simulink subsystem "FanModule_2025a"  (R2026a)
settings: Solver=VariableStepAuto
model mask{min_fan_speed=0.05, tau=0.1, max_thrust=3.53, radius=0.5, max_speed=62500}
  mask prompts: min_fan_speed "min Fan Speed (%)"; tau "Time Constant (s)"; max_thrust "Max Thrust (N)"; radius "Radius (m)"; max_speed "Max Speed (RPM)"
undefined symbols (not defined in the file): IN
settings Model: Creator=wangzerun  LastModifiedBy=asing

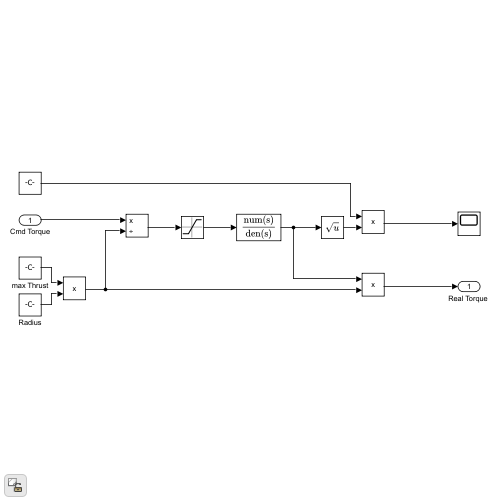
[thumbnail: Simulink's stored preview of the top-level diagram]
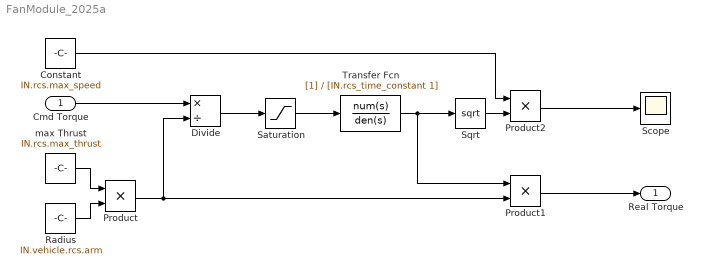
== system FanModule_2025a ==
  Cmd Torque : Inport
  Constant : Constant  Value=IN.rcs.max_speed
  Divide : Product  Inputs=*/
  Product : Product
  Product1 : Product
  Product2 : Product
  Radius : Constant  Value=IN.vehicle.rcs.arm
  Saturation : Saturate  UpperLimit=1  LowerLimit=IN.rcs.min_speed
  Scope : Scope
  Sqrt : Sqrt
  Transfer Fcn : TransferFcn  Denominator=[IN.rcs_time_constant 1]
  max Thrust : Constant  Value=IN.rcs.max_thrust
  "Real Torque " : Outport
  wires:
  Transfer Fcn/1 -> Sqrt/1, Product1/1
  Saturation/1 -> Transfer Fcn/1
  Cmd Torque/1 -> Divide/1
  Divide/1 -> Saturation/1
  max Thrust/1 -> Product/1
  Radius/1 -> Product/2
  Product/1 -> Product1/2, Divide/2
  Product1/1 -> "Real Torque "/1
  Sqrt/1 -> Product2/2
  Constant/1 -> Product2/1
  Product2/1 -> Scope/1
